simulink model "walking_beam"  (R2026a)
settings: Solver=daessc  StopTime=5  MaxStep=5e-4  RelTol=1e-4
StopFcn:
  | plot_F3_vs_theta2
values from neighbouring files (symbols this model uses):
  s = sign(v)    [plot_F3_vs_theta2.m]
undefined symbols (not defined in the file or in its folder): X, Y, Z
libraries: sm_lib x33, nesl_utility x10, simulink x1
(part 1 of 2)
settings Model: Creator=Admin  LastModifiedBy=Admin
settings SimscapeCC: SimscapeLogType=none
settings ExplorerConfigSet: InternalSimMechanicsExplorerSettings=|
  | <ExplorerConfiguration>
  | 
  |   <canonicalview>default</canonicalview>
  | 
  |   <TilePanel>
  |     <TileInfo>
  |       <Tiles Columns="1" Count="1" Height="706" Rows="1" Width="1316">
  |         <Row Weight="1"/>
  |         <Column Weight="1"/>
  |         <Tile Height="1" Width="1" X="0" Y="0"/>
  |       </Tiles>
  |     </TileInfo>
  |     <SceneInfo>
  |       <SceneViewer>
  |         <IsThisViewStd>
  |           <IsStandardView>off</IsStandardView>
  |           <StandardViewName>Front</StandardViewName>
  |         </IsThisViewStd>
  |         <BGColor>
  |           <R>1</R>
  |           <G>1</G>
  |           <B>1</B>
  |           <A>1</A>
  |         </BGColor>
  |         <Camera>
  |           <DoPerspective>off</DoPerspective>
  |           <Position>
  |             <X>0.069016977308352018</X>
  |             <Y>-0.1702544305806459</Y>
  |             <Z>1.192738584381912</Z>
  |           </Position>
  |           <Center>
  |             <X>0.29948564897094587</X>
  |             <Y>0.074994979776969922</Y>
  |             <Z>0.089914238686012116</Z>
  |           </Center>
  |           <Up>
  |             <X>0.10827439580495295</X>
  |             <Y>0.9653807046978804</Y>
  |             <Z>0.23731150458858177</Z>
  |           </Up>
  |           <XLim>0.16957681948984568</XLim>
  |           <YLim>0.16957681948984568</YLim>
  |           <ViewLimDist>0.01</ViewLimDist>
  |         </Camera>
  |       </SceneViewer>
  |     </SceneInfo>
  |   </TilePanel>
  | 
  |   <MechEditorPanel>
  |     <GfxPanelCameraMap/>
  |     <Cameras/>
  |     <VideoCreator>
  |       <IncludeTiles>All</IncludeTiles>
  |       <IncludeTime>on</IncludeTime>
  |       <IncludeWorldFrame>off</IncludeWorldFrame>
  |       <PlaybackSpeedRatio>1</PlaybackSpeedRatio>
  |       <FrameRate>60</FrameRate>
  |       <FrameSize>auto</FrameSize>
  |       <VideoFormat>MotionJPEGAVI</VideoFormat>
  |     </VideoCreator>
  |   </MechEditorPanel>
  | 
  |   <PlaybackSettings>
  |     <PlaybackSpeedFactor>1</PlaybackSpeedFactor>
  |   </PlaybackSettings>
  | 
  | </ExplorerConfiguration>

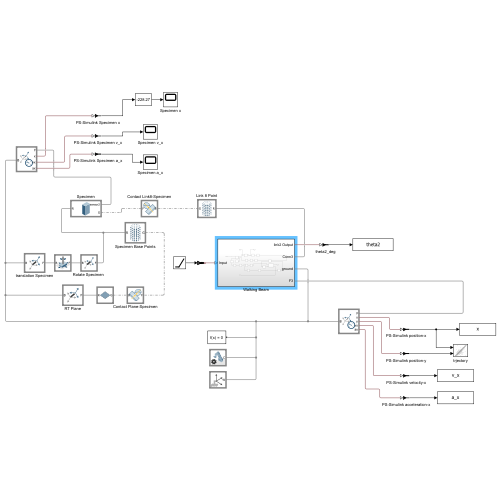
[thumbnail: Simulink's stored preview of the top-level diagram]
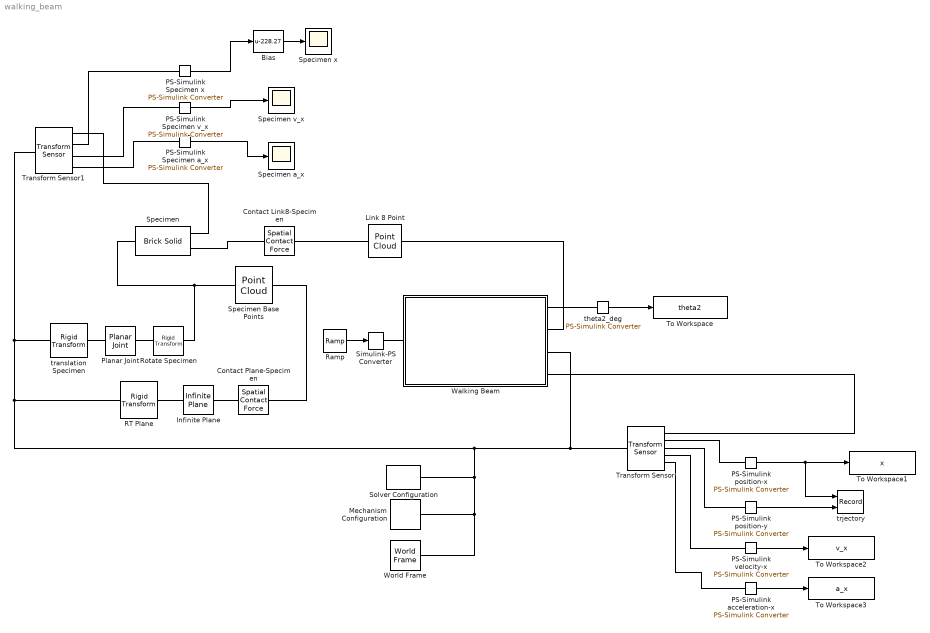
== system walking_beam ==
  Bias : Bias  Bias=-228.27  SaturateOnIntegerOverflow=off
  Contact Link8-Specimen : sm_lib/Forces and Torques/Spatial Contact Force  SenseSeparationDistance=off  NormalForceType=SmoothSpringDamper  NormalStiffness=500  NormalStiffnessUnits=N/m  NormalDamping=1.4  NormalDampingUnits=N/(m/s)  NormalTransitionRegionWidth=1e-05  NormalTransitionRegionWidthUnits=m  FrictionType=SmoothStickSlip  CoefficientOfStaticFriction=0.4  CoefficientOfDynamicFriction=0.3  FrictionalCriticalVelocity=0.001  FrictionalCriticalVelocityUnits=m/s  SenseContactSignal=off  SensePenetrationDepth=off  SenseNormalVelocity=off  SenseTangentialVelocity=off  SensingForceTorqueDirection=BaseOnFollower  SensingForceTorqueResolutionFrame=BaseFrame  SenseNormalForce=off  SenseNormalForceMagnitude=off  SenseNormalTorque=off  SenseFrictionalForce=off  SenseFrictionalForceMagnitude=off  SenseFrictionalTorque=off  SenseTotalForce=off  SenseTotalTorque=off  SenseContactBaseRotation=off  SenseContactBaseTranslation=off  SenseContactFollowerRotation=off  SenseContactFollowerTranslation=off  ZeroCrossDetectContactStartAndEnd=off
  Contact Plane-Specimen : sm_lib/Forces and Torques/Spatial Contact Force  SenseSeparationDistance=off  NormalForceType=SmoothSpringDamper  NormalStiffness=500  NormalStiffnessUnits=N/m  NormalDamping=0.7  NormalDampingUnits=N/(m/s)  NormalTransitionRegionWidth=1e-05  NormalTransitionRegionWidthUnits=m  FrictionType=SmoothStickSlip  CoefficientOfStaticFriction=0.4  CoefficientOfDynamicFriction=0.3  FrictionalCriticalVelocity=0.001  FrictionalCriticalVelocityUnits=m/s  SenseContactSignal=off  SensePenetrationDepth=off  SenseNormalVelocity=off  SenseTangentialVelocity=off  SensingForceTorqueDirection=BaseOnFollower  SensingForceTorqueResolutionFrame=BaseFrame  SenseNormalForce=off  SenseNormalForceMagnitude=off  SenseNormalTorque=off  SenseFrictionalForce=off  SenseFrictionalForceMagnitude=off  SenseFrictionalTorque=off  SenseTotalForce=off  SenseTotalTorque=off  SenseContactBaseRotation=off  SenseContactBaseTranslation=off  SenseContactFollowerRotation=off  SenseContactFollowerTranslation=off  ZeroCrossDetectContactStartAndEnd=off
  Infinite Plane : sm_lib/Curves and Surfaces/Infinite Plane  GraphicType=Rectangle  GraphicPlaneWidth=300  GraphicPlaneWidthUnits=mm  GraphicPlaneHeight=60  GraphicPlaneHeightUnits=mm  GraphicVisPropType=SimpleVisualProperties  GraphicDiffuseColor=[1 1 1]  GraphicOpacity=0  GraphicSpecularColor=[0.5 0.5 0.5 1.0]  GraphicAmbientColor=[0.15 0.15 0.15 1.0]  GraphicEmissiveColor=[0.0 0.0 0.0 1.0]  GraphicShininess=75
  Link 8 Point : sm_lib/Curves and Surfaces/Point Cloud  CoordinatesMatrix=[-16.663 2.5 -98.537;-16.663 2.5 -97.5701;-16.663 2.5 -96.6031;-16.663 2.5 -95.6362;-16.663 2.5 -94.6693;-16.663 2.5 -93.7024;-16.663 2.5 -92.7354;-16.663 2.5 -91.7685;-16.663 2.5 -90.8016;-16.663 2.5 -89.8346;-16.663 2.5 -88.8677;-16.663 2.5 -87.9008;-16.663 2.5 -86.9339;-16.663 2.5 -85.9669;-16.663 2.5 -85;-15.663 2.5 -98.537;-14.663 2.5 -98.537;-14.663 2.5 -97.5701;-14.663 2.5 -96.6031;-14.663 2.5 -95.6362;-14.663 2.5 -94.6693;-14.663 2.5 -93.7024;-14.663 2.5 -92.7354;-14.663 2.5 -91.7685;-14.663 2.5 -90.8016;-14.663 2.5 -89.8346;-14.663 2.5 -88.8677;-14.663 2.5 -87.9008;-14.663 2.5 -86.9339;-14.663 2.5 -85.9669;-14.663 2.5 -85;0.337 2.5 -98.537;0.337 2.5 -97.5701;0.337 2.5 -96.6031;0.337 2.5 -95.6362;0.337 2.5 -94.6693;0.337 2.5 -93.7024;0.337 2.5 -92.7354;0.337 2.5 -91.7685;0.337 2.5 -90.8016;0.337 2.5 -89.8346;0.337 2.5 -88.8677;0.337 2.5 -87.9008;0.337 2.5 -86.9339;0.337 2.5 -85.9669;0.337 2.5 -85;1.337 2.5 -98.537;2.337 2.5 -98.537;2.337 2.5 -97.5701;2.337 2.5 -96.6031;2.337 2.5 -95.6362;2.337 2.5 -94.6693;2.337 2.5 -93.7024;2.337 2.5 -92.7354;2.337 2.5 -91.7685;2.337 2.5 -90.8016;2.337 2.5 -89.8346;2.337 2.5 -88.8677;2.337 2.5 -87.9008;2.337 2.5 -86.9339;2.337 2.5 -85.9669;2.337 2.5 -85;17.337 2.5 -98.537;17.337 2.5 -97.5701;17.337 2.5 -96.6031;17.337 2.5 -95.6362;17.337 2.5 -94.6693;17.337 2.5 -93.7024;17.337 2.5 -92.7354;17.337 2.5 -91.7685;17.337 2.5 -90.8016;17.337 2.5 -89.8346;17.337 2.5 -88.8677;17.337 2.5 -87.9008;17.337 2.5 -86.9339;17.337 2.5 -85.9669;17.337 2.5 -85;18.337 2.5 -98.537;19.337 2.5 -98.537;19.337 2.5 -97.5701;19.337 2.5 -96.6031;19.337 2.5 -95.6362;19.337 2.5 -94.6693;19.337 2.5 -93.7024;19.337 2.5 -92.7354;19.337 2.5 -91.7685;19.337 2.5 -90.8016;19.337 2.5 -89.8346;19.337 2.5 -88.8677;19.337 2.5 -87.9008;19.337 2.5 -86.9339;19.337 2.5 -85.9669;19.337 2.5 -85;34.337 2.5 -98.537;34.337 2.5 -97.5701;34.337 2.5 -96.6031;34.337 2.5 -95.6362;34.337 2.5 -94.6693;34.337 2.5 -93.7024;34.337 2.5 -92.7354;34.337 2.5 -91.7685;34.337 2.5 -90.8016;34.337 2.5 -89.8346;34.337 2.5 -88.8677;34.337 2.5 -87.9008;34.337 2.5 -86.9339;34.337 2.5 -85.9669;34.337 2.5 -85;35.337 2.5 -98.537;36.337 2.5 -98.537;36.337 2.5 -97.5701;36.337 2.5 -96.6031;36.337 2.5 -95.6362;36.337 2.5 -94.6693;36.337 2.5 -93.7024;36.337 2.5 -92.7354;36.337 2.5 -91.7685;36.337 2.5 -90.8016;36.337 2.5 -89.8346;36.337 2.5 -88.8677;36.337 2.5 -87.9008;36.337 2.5 -86.9339;36.337 2.5 -85.9669;36.337 2.5 -85;51.337 2.5 -98.537;51.337 2.5 -97.5701;51.337 2.5 -96.6031;51.337 2.5 -95.6362;51.337 2.5 -94.6693;51.337 2.5 -93.7024;51.337 2.5 -92.7354;51.337 2.5 -91.7685;51.337 2.5 -90.8016;51.337 2.5 -89.8346;51.337 2.5 -88.8677;51.337 2.5 -87.9008;51.337 2.5 -86.9339;51.337 2.5 -85.9669;51.337 2.5 -85;52.337 2.5 -98.537;53.337 2.5 -98.537;53.337 2.5 -97.5701;53.337 2.5 -96.6031;53.337 2.5 -95.6362;53.337 2.5 -94.6693;53.337 2.5 -93.7024;53.337 2.5 -92.7354;53.337 2.5 -91.7685;53.337 2.5 -90.8016;53.337 2.5 -89.8346;53.337 2.5 -88.8677;53.337 2.5 -87.9008;53.337 2.5 -86.9339;53.337 2.5 -85.9669;53.337 2.5 -85;68.337 2.5 -98.537;68.337 2.5 -97.5701;68.337 2.5 -96.6031;68.337 2.5 -95.6362;68.337 2.5 -94.6693;68.337 2.5 -93.7024;68.337 2.5 -92.7354;68.337 2.5 -91.7685;68.337 2.5 -90.8016;68.337 2.5 -89.8346;68.337 2.5 -88.8677;68.337 2.5 -87.9008;68.337 2.5 -86.9339;68.337 2.5 -85.9669;68.337 2.5 -85;69.337 2.5 -98.537;70.337 2.5 -98.537;70.337 2.5 -97.5701;70.337 2.5 -96.6031;70.337 2.5 -95.6362;70.337 2.5 -94.6693;70.337 2.5 -93.7024;70.337 2.5 -92.7354;70.337 2.5 -91.7685;70.337 2.5 -90.8016;70.337 2.5 -89.8346;70.337 2.5 -88.8677;70.337 2.5 -87.9008;70.337 2.5 -86.9339;70.337 2.5 -85.9669;70.337 2.5 -85;85.337 2.5 -98.537;85.337 2.5 -97.5701;85.337 2.5 -96.6031;85.337 2.5 -95.6362;85.337 2.5 -94.6693;85.337 2.5 -93.7024;85.337 2.5 -92.7354;85.337 2.5 -91.7685;85.337 2.5 -90.8016;85.337 2.5 -89.8346;85.337 2.5 -88.8677;85.337 2.5 -87.9008;85.337 2.5 -86.9339;85.337 2.5 -85.9669;85.337 2.5 -85;86.337 2.5 -98.537;87.337 2.5 -98.537;87.337 2.5 -97.5701 ...(+3445 chars)]  CoordinatesMatrixUnits=mm  GraphicType=MarkerCloud  GraphicSphereRadius=0.4  GraphicSphereRadiusUnits=mm  GraphicVisPropType=SimpleVisualProperties  GraphicDiffuseColor=[0.9 0.1 0.1]  GraphicOpacity=1  GraphicSpecularColor=[0.5 0.5 0.5 1.0]  GraphicAmbientColor=[0.15 0.15 0.15 1.0]  GraphicEmissiveColor=[0.0 0.0 0.0 1.0]  GraphicShininess=75
  Mechanism Configuration : sm_lib/Utilities/Mechanism Configuration  UniformGravity=Constant  GravityVector=[0 -9.80665 0]  GravityVectorUnits=m/s^2  LinearizationDelta=0.001  JointModeTransitionNonlinearIterations=2
  PS-Simulink Specimen a_x : nesl_utility/PS-Simulink Converter  PhysicalDomain=network_engine_domain  SubClassName=ps_output  LeftPortType=input  RightPortType=output  PseudoPeriodic=off  Frequencies=[]  VectorFormat=1-D array  Unit=mm/s^2  AffineConversion=off
  PS-Simulink Specimen v_x : nesl_utility/PS-Simulink Converter  PhysicalDomain=network_engine_domain  SubClassName=ps_output  LeftPortType=input  RightPortType=output  PseudoPeriodic=off  Frequencies=[]  VectorFormat=1-D array  Unit=mm/s  AffineConversion=off
  PS-Simulink Specimen x : nesl_utility/PS-Simulink Converter  PhysicalDomain=network_engine_domain  SubClassName=ps_output  LeftPortType=input  RightPortType=output  PseudoPeriodic=off  Frequencies=[]  VectorFormat=1-D array  Unit=mm  AffineConversion=off
  PS-Simulink acceleration-x : nesl_utility/PS-Simulink Converter  PhysicalDomain=network_engine_domain  SubClassName=ps_output  LeftPortType=input  RightPortType=output  PseudoPeriodic=off  Frequencies=[]  VectorFormat=inherit  Unit=mm/s^2  AffineConversion=off
  PS-Simulink position-x : nesl_utility/PS-Simulink Converter  PhysicalDomain=network_engine_domain  SubClassName=ps_output  LeftPortType=input  RightPortType=output  PseudoPeriodic=off  Frequencies=[]  VectorFormat=1-D array  Unit=mm  AffineConversion=off
  PS-Simulink position-y : nesl_utility/PS-Simulink Converter  PhysicalDomain=network_engine_domain  SubClassName=ps_output  LeftPortType=input  RightPortType=output  PseudoPeriodic=off  Frequencies=[]  VectorFormat=1-D array  Unit=mm  AffineConversion=off
  PS-Simulink velocity-x : nesl_utility/PS-Simulink Converter  PhysicalDomain=network_engine_domain  SubClassName=ps_output  LeftPortType=input  RightPortType=output  PseudoPeriodic=off  Frequencies=[]  VectorFormat=inherit  Unit=mm/s  AffineConversion=off
  Planar Joint : sm_lib/Joints/Planar Joint  JointMode=Normal  CompositeWrenchDir=FollowerOnBase  CompositeWrenchFrame=BaseFrame  SenseConstraintForce=off  SenseConstraintTorque=off  SenseTotalForce=off  SenseTotalTorque=off  PxPositionTargetSpecify=on  PxPositionTargetPriority=High  PxPositionTargetValue=228.27  PxPositionTargetValueUnits=mm  PxVelocityTargetSpecify=on  PxVelocityTargetPriority=High  PxVelocityTargetValue=0  PxVelocityTargetValueUnits=m/s  PxEquilibriumPosition=0  PxEquilibriumPositionUnits=m  PxSpringStiffness=0  PxSpringStiffnessUnits=N/m  PxDampingCoefficient=0  PxDampingCoefficientUnits=N/(m/s)  PxLowerLimitSpecify=off  PxLowerLimitBound=-1  PxLowerLimitBoundUnits=m  PxLowerLimitStiffness=1e6  PxLowerLimitStiffnessUnits=N/m  PxLowerLimitDamping=1e3  PxLowerLimitDampingUnits=N/(m/s)  PxLowerLimitTransitionRegionWidth=1e-4  PxLowerLimitTransitionRegionWidthUnits=m  PxUpperLimitSpecify=off  PxUpperLimitBound=1  PxUpperLimitBoundUnits=m  PxUpperLimitStiffness=1e6  PxUpperLimitStiffnessUnits=N/m  PxUpperLimitDamping=1e3  PxUpperLimitDampingUnits=N/(m/s)  PxUpperLimitTransitionRegionWidth=1e-4  PxUpperLimitTransitionRegionWidthUnits=m  PxTorqueActuationMode=NoTorque  PxMotionActuationMode=ComputedMotion  PxSensePosition=off  PxSenseVelocity=off  PxSenseAcceleration=off  PxSenseTorqueForce=off  PxSenseLowerLimitTorqueForce=off  PxSenseUpperLimitTorqueForce=off  PyPositionTargetSpecify=on  PyPositionTargetPriority=High  PyPositionTargetValue=187.1  PyPositionTargetValueUnits=mm  PyVelocityTargetSpecify=on  PyVelocityTargetPriority=High  PyVelocityTargetValue=0  PyVelocityTargetValueUnits=m/s  PyEquilibriumPosition=0  PyEquilibriumPositionUnits=m  PySpringStiffness=0  PySpringStiffnessUnits=N/m  PyDampingCoefficient=0  PyDampingCoefficientUnits=N/(m/s)  PyLowerLimitSpecify=off  PyLowerLimitBound=-1  PyLowerLimitBoundUnits=m  PyLowerLimitStiffness=1e6  PyLowerLimitStiffnessUnits=N/m  PyLowerLimitDamping=1e3  PyLowerLimitDampingUnits=N/(m/s)  PyLowerLimitTransitionRegionWidth=1e-4  PyLowerLimitTransitionRegionWidthUnits=m  PyUpperLimitSpecify=off  PyUpperLimitBound=1  PyUpperLimitBoundUnits=m  PyUpperLimitStiffness=1e6  PyUpperLimitStiffnessUnits=N/m  PyUpperLimitDamping=1e3  PyUpperLimitDampingUnits=N/(m/s)  PyUpperLimitTransitionRegionWidth=1e-4  PyUpperLimitTransitionRegionWidthUnits=m  PyTorqueActuationMode=NoTorque  PyMotionActuationMode=ComputedMotion  PySensePosition=off  PySenseVelocity=off  PySenseAcceleration=off  PySenseTorqueForce=off  PySenseLowerLimitTorqueForce=off  PySenseUpperLimitTorqueForce=off  RzPositionTargetSpecify=on  RzPositionTargetPriority=High  RzPositionTargetValue=0  RzPositionTargetValueUnits=deg  RzVelocityTargetSpecify=on  RzVelocityTargetPriority=High  RzVelocityTargetValue=0  RzVelocityTargetValueUnits=deg/s  RzEquilibriumPosition=0  RzEquilibriumPositionUnits=deg  RzSpringStiffness=0  RzSpringStiffnessUnits=N*m/deg  RzDampingCoefficient=0  RzDampingCoefficientUnits=N*m/(deg/s)  RzLowerLimitSpecify=off  RzLowerLimitBound=-90  RzLowerLimitBoundUnits=deg  RzLowerLimitStiffness=1e4  RzLowerLimitStiffnessUnits=N*m/deg  RzLowerLimitDamping=10  RzLowerLimitDampingUnits=N*m/(deg/s)  RzLowerLimitTransitionRegionWidth=0.1  RzLowerLimitTransitionRegionWidthUnits=deg  RzUpperLimitSpecify=off  RzUpperLimitBound=90  RzUpperLimitBoundUnits=deg  RzUpperLimitStiffness=1e4  RzUpperLimitStiffnessUnits=N*m/deg  RzUpperLimitDamping=10  RzUpperLimitDampingUnits=N*m/(deg/s)  RzUpperLimitTransitionRegionWidth=0.1  RzUpperLimitTransitionRegionWidthUnits=deg  RzTorqueActuationMode=NoTorque  RzMotionActuationMode=ComputedMotion  RzSensePosition=off  RzSenseVelocity=off  RzSenseAcceleration=off  RzSenseTorqueForce=off  RzSenseLowerLimitTorqueForce=off  RzSenseUpperLimitTorqueForce=off
  RT Plane : sm_lib/Frames and Transforms/Rigid Transform  RotationMethod=StandardAxis  FollAlignAxisA=+X  BaseAlignAxisA=+Y  FollAlignAxisB=+Y  BaseAlignAxisB=+Z  RotationStandardAxis=+X  RotationAngle=-90  RotationAngleUnits=deg  RotationArbitraryAxis=[0 0 1]  RotationSequenceAxes=FollowerAxes  RotationSequence=XYX  RotationSequenceAngles=[0 0 0]  RotationSequenceAnglesUnits=deg  RotationMatrix=[1 0 0;0 1 0;0 0 1]  Quaternion=[1 0 0 0]  TranslationMethod=Cartesian  TranslationCartesianOffset=[228.27 184.6 128.77]  TranslationCartesianOffsetUnits=mm  TranslationStandardAxis=+Z  TranslationStandardOffset=0  TranslationStandardOffsetUnits=m  TranslationROffset=0  TranslationROffsetUnits=m  TranslationThetaOffset=0  TranslationThetaOffsetUnits=deg  TranslationZOffset=0  TranslationZOffsetUnits=m
  Ramp : simulink/Sources/Ramp  slope=10  start=0  InitialOutput=10
  "Rotate Specimen " : sm_lib/Frames and Transforms/Rigid Transform  RotationMethod=StandardAxis  FollAlignAxisA=+X  BaseAlignAxisA=+Y  FollAlignAxisB=+Y  BaseAlignAxisB=+Z  RotationStandardAxis=+X  RotationAngle=90  RotationAngleUnits=deg  RotationArbitraryAxis=[0 0 1]  RotationSequenceAxes=FollowerAxes  RotationSequence=XYX  RotationSequenceAngles=[0 0 0]  RotationSequenceAnglesUnits=deg  RotationMatrix=[1 0 0;0 1 0;0 0 1]  Quaternion=[1 0 0 0]  TranslationMethod=None  TranslationCartesianOffset=[0 0 0]  TranslationCartesianOffsetUnits=m  TranslationStandardAxis=+Z  TranslationStandardOffset=0  TranslationStandardOffsetUnits=m  TranslationROffset=0  TranslationROffsetUnits=m  TranslationThetaOffset=0  TranslationThetaOffsetUnits=deg  TranslationZOffset=0  TranslationZOffsetUnits=m
  Simulink-PS Converter : nesl_utility/Simulink-PS Converter  PhysicalDomain=network_engine_domain  SubClassName=ps_input  LeftPortType=input  RightPortType=output  PseudoPeriodic=off  Frequencies=[]  NoiseDistribution=none  NoiseParameters=[]  Unit=rad  AffineConversion=off  FilteringAndDerivatives=filter  SimscapeFilterOrder=2  InputFilterTimeConstant=0.001  UdotUserProvided=0
  Solver Configuration : nesl_utility/Solver Configuration  PhysicalDomain=network_engine_domain  SubClassName=solver  LeftPortType=input  RightPortType=generic  Tones=[]  Harmonics=[]  SimulateNoise=off  Profile=off  UseLocalSampling=off  EnableSwitchedLinearOptims=on  FrequencyDomain=off  UseCCode=off  RelTol=0.001  AbsTol=0.001  MinStep=1e-09  ToWorkspace=off  RevertToSquareIcSolve=off  NumHomotopyIterations=100  PhasorMode=off  PhasorModeNumHarmonics=1  ConsistencySolver=NEWTON_XTOL_AFTER_FTOL  CanonicalOrdering=CANONICAL  OptimizeIntermediates=OPTIMIZED  IndexReductionMethod=DerivativeReplacement  DoDC=off  ResidualTolerance=1e-09  ConsistencyTolSource=GLOBAL  ConsistencyAbsTol=0.001  ConsistencyRelTol=0.001  ConsistencyTolFactor=0.001  UseLocalSolver=off  LocalSolverChoice=NE_BACKWARD_EULER_ADVANCER  ResolveIndetEquations=on  FunctionEvalNumThread=1  LocalSolverSampleTime=0.001  DoFixedCost=off  MaxNonlinIter=3  MaxModeIter=2  ComputeImpulses=off  ImpulseIterations=2  LinearAlgebra=auto  LinearAlgebraNumThread=0  EquationFormulation=NE_TIME_EF  DelaysMemoryBudget=1024  AutomaticFiltering=on  FilteringTimeConstant=0.001  PartitionStorageMethod=AS_NEEDED  PartitionMemoryBudget=1024  PartitionMethod=ROBUST  MultibodyUseLocalSolver=off  MultibodyLocalSolverChoice=ODE1  MultibodyLocalSolverSampleTime=0.001
  Specimen : sm_lib/Body Elements/Brick Solid  BrickDimensions=[5 30 5]  BrickDimensionsUnits=mm  ExportEntireGeometry=on  InertiaType=CalculateFromGeometry  BasedOnType=Density  Density=1000  DensityUnits=kg/m^3  Mass=1  MassUnits=kg  CenterOfMass=[0 0 0]  CenterOfMassUnits=m  MomentsOfInertia=[1 1 1]  MomentsOfInertiaUnits=kg*m^2  ProductsOfInertia=[0 0 0]  ProductsOfInertiaUnits=kg*m^2  GraphicType=FromGeometry  MarkerShape=Sphere  MarkerSize=10  GraphicVisPropType=SimpleVisualProperties  GraphicDiffuseColor=[0.75 0.65 0.95]  GraphicOpacity=1  GraphicSpecularColor=[0.5 0.5 0.5 1.0]  GraphicAmbientColor=[0.15 0.15 0.15 1.0]  GraphicEmissiveColor=[0.0 0.0 0.0 1.0]  GraphicShininess=75  DoExposeReferenceFrame=on  SerializedFrames=|
      | <Frames>
      | 
      |   <Frame>
      |     <Id>Frame1</Id>
      |     <Value>
      |       <Name>sensor2</Name>
      |       <Origin>
      |         <Source>ReferenceFrame</Source>
      |         <FeatureName></FeatureName>
      |       </Origin>
      |       <PrimaryAxis>
      |         <DefinedDirection>+Z</DefinedDirection>
      |         <Source>ReferenceFrame</Source>
      |         <SourceDirection>+Z</SourceDirection>
      |         <FeatureName></FeatureName>
      |       </PrimaryAxis>
      |       <SecondaryAxis>
      |         <DefinedDirection>+X</DefinedDirection>
      |         <Source>ReferenceFrame</Source>
      |         <SourceDirection>+X</SourceDirection>
      |         <FeatureName></FeatureName>
      |       </SecondaryAxis>
      |     </Value>
      |   </Frame>
      | 
      | </Frames>
  Specimen Base Points : sm_lib/Curves and Surfaces/Point Cloud  CoordinatesMatrix=[-2.5 -10 2.5;2.5 -10 2.5;2.5 10 2.5;-2.5 10 2.5]  CoordinatesMatrixUnits=mm  GraphicType=MarkerCloud  GraphicSphereRadius=0.4  GraphicSphereRadiusUnits=mm  GraphicVisPropType=SimpleVisualProperties  GraphicDiffuseColor=[0.2 0.2 0.9]  GraphicOpacity=1  GraphicSpecularColor=[0.5 0.5 0.5 1.0]  GraphicAmbientColor=[0.15 0.15 0.15 1.0]  GraphicEmissiveColor=[0.0 0.0 0.0 1.0]  GraphicShininess=75
  Specimen a_x : Scope
      settings: ActiveDisplayYMinimum=-128615.45700333494  ActiveDisplayYMaximum=1.0858097042017304E+6  DataLoggingVariableName=ScopeData2
  Specimen v_x : Scope
      settings: ActiveDisplayYMinimum=-17.214449819310651  ActiveDisplayYMaximum=151.84850866140505
  Specimen x : Scope
      settings: ActiveDisplayYMinimum=-28.751888500285233  ActiveDisplayYMaximum=165.83973606812339
  To Workspace : ToWorkspace  VariableName=theta2  SaveFormat=Timeseries  SampleTime=-1
  To Workspace1 : ToWorkspace  VariableName=x  SaveFormat=Timeseries  SampleTime=-1
  To Workspace2 : ToWorkspace  VariableName=v_x  SaveFormat=Timeseries  SampleTime=-1
  To Workspace3 : ToWorkspace  VariableName=a_x  SaveFormat=Timeseries  SampleTime=-1
  Transform Sensor : sm_lib/Frames and Transforms/Transform Sensor  MeasurementFrame=World  RotationSequence=XYX  SenseAngle=off  SenseAxis=off  SenseQ=off  SenseR=off  SenseRotationSequence=off  SenseOmegaX=off  SenseOmegaY=off  SenseOmegaZ=off  SenseOmega=off  SenseQDot=off  SenseRDot=off  SenseRotationSequenceDot=off  SenseAlphaX=off  SenseAlphaY=off  SenseAlphaZ=off  SenseAlpha=off  SenseQDDot=off  SenseRDDot=off  SenseX=on  SenseY=on  SenseZ=off  SenseXYZ=off  SenseRad=off  SenseAzim=off  SenseDist=off  SenseInc=off  SenseXDot=on  SenseYDot=off  SenseZDot=off  SenseXYZDot=off  SenseRadDot=off  SenseAzimDot=off  SenseDistDot=off  SenseIncDot=off  SenseXDDot=on  SenseYDDot=off  SenseZDDot=off  SenseXYZDDot=off  SenseRadDDot=off  SenseAzimDDot=off  SenseDistDDot=off  SenseIncDDot=off
  Transform Sensor1 : sm_lib/Frames and Transforms/Transform Sensor  MeasurementFrame=World  RotationSequence=XYX  SenseAngle=off  SenseAxis=off  SenseQ=off  SenseR=off  SenseRotationSequence=off  SenseOmegaX=off  SenseOmegaY=off  SenseOmegaZ=off  SenseOmega=off  SenseQDot=off  SenseRDot=off  SenseRotationSequenceDot=off  SenseAlphaX=off  SenseAlphaY=off  SenseAlphaZ=off  SenseAlpha=off  SenseQDDot=off  SenseRDDot=off  SenseX=on  SenseY=off  SenseZ=off  SenseXYZ=off  SenseRad=off  SenseAzim=off  SenseDist=off  SenseInc=off  SenseXDot=on  SenseYDot=off  SenseZDot=off  SenseXYZDot=off  SenseRadDot=off  SenseAzimDot=off  SenseDistDot=off  SenseIncDot=off  SenseXDDot=on  SenseYDDot=off  SenseZDDot=off  SenseXYZDDot=off  SenseRadDDot=off  SenseAzimDDot=off  SenseDistDDot=off  SenseIncDDot=off
  Walking Beam : Subsystem
  World Frame : sm_lib/Frames and Transforms/World Frame
  theta2_deg : nesl_utility/PS-Simulink Converter  PhysicalDomain=network_engine_domain  SubClassName=ps_output  LeftPortType=input  RightPortType=output  PseudoPeriodic=off  Frequencies=[]  VectorFormat=1-D array  Unit=deg  AffineConversion=off
  translation Specimen : sm_lib/Frames and Transforms/Rigid Transform  RotationMethod=None  FollAlignAxisA=+X  BaseAlignAxisA=+Y  FollAlignAxisB=+Y  BaseAlignAxisB=+Z  RotationStandardAxis=+Z  RotationAngle=0  RotationAngleUnits=deg  RotationArbitraryAxis=[0 0 1]  RotationSequenceAxes=FollowerAxes  RotationSequence=XYX  RotationSequenceAngles=[0 0 0]  RotationSequenceAnglesUnits=deg  RotationMatrix=[1 0 0;0 1 0;0 0 1]  Quaternion=[1 0 0 0]  TranslationMethod=Cartesian  TranslationCartesianOffset=[0 0 128.77]  TranslationCartesianOffsetUnits=mm  TranslationStandardAxis=+Z  TranslationStandardOffset=0  TranslationStandardOffsetUnits=m  TranslationROffset=0  TranslationROffsetUnits=m  TranslationThetaOffset=0  TranslationThetaOffsetUnits=deg  TranslationZOffset=0  TranslationZOffsetUnits=m
  trjectory : Record  NumPorts=2.0  FileSettingsInternal="{\"entries\":[{\"content\":{\"excelSettings\":{\"content\":{},\"type\":\"Streamout.ExcelSettings\"},\"parquetSettings\":{\"content\":{},\"type\":\"Streamout.ParquetSettings\"}},\"type\":\"Streamout.FileSettingStorage\",\"uuid\":\"\"}],\"packageUris\":[\"http:\\/\\/schema.mathworks.com\\/mf0\\/streamout_blocks\\/R2020a\"],\"version\":\"1.0\"}"  FrameSettings=[0, 0]  Layout=[1 1]  SignalsInternal="{\"entries\":[{\"content\":{\"signals\":[{\"content\":{\"blockPath\":[],\"dimensions\":[1],\"domain\":\"\",\"lineColor\":\"#fe330a\",\"lineWidth\":2,\"plots\":[ 1 ],\"port\":1,\"sid\":[\"\"],\"signalID\":1,\"signalName\":\"PS-Simulink position-x\"},\"type\":\"RecordBlkView.Signal\",\"uuid\":\"\"},{\"content\":{\"blockPath\":[],\"dimensions\":[1],\"domain\":\"\",\"lineColor\":\"#139fff\",\"plots\":[ 1 ],\"port\":2,\"sid\":[\"\"],\"signalID\":2,\"signalName\":\"PS-Simulink position-y\"},\"type\":\"RecordBlkView.Signal\",\"uuid\":\"\"}]},\"type\":\"RecordBlkView.InputSignals\",\"uuid\":\"\"}],\"packageUris\":[\"http:\\/\\/schema.mathworks.com\\/mf0\\/streamout_blocks\\/R2020a\"],\"version\":\"1.0\"}"  VisualizationBindings="{\"xyplotplugin\":{\"info\":[{\"series\":[{\"bindingParametersList\":[{\"parameter\":\"X-Axis\",\"signalID\":1,\"signalName\":\"PS-Simulink position-x\"},{\"parameter\":\"Y-Axis\",\"signalID\":2,\"signalName\":\"PS-Simulink position-y\"}],\"seriesID\":0}],\"subplotID\":1}]}}"  CompatibilityTag=XY
  wires:
  Ramp/1 -> Simulink-PS Converter/1
  PS-Simulink position-x/1 -> To Workspace1/1, trjectory/1
  PS-Simulink position-y/1 -> trjectory/2
  theta2_deg/1 -> To Workspace/1
  PS-Simulink velocity-x/1 -> To Workspace2/1
  PS-Simulink acceleration-x/1 -> To Workspace3/1
  PS-Simulink Specimen x/1 -> Bias/1
  PS-Simulink Specimen v_x/1 -> Specimen v_x/1
  PS-Simulink Specimen a_x/1 -> Specimen a_x/1
  Bias/1 -> Specimen x/1
  connections:
  Solver Configuration/RConn1 -- Walking Beam/RConn3 -- Transform Sensor/LConn1 -- Transform Sensor1/LConn1 -- translation Specimen/LConn1 -- RT Plane/LConn1 -- World Frame/RConn1 -- Mechanism Configuration/RConn1
  PS-Simulink position-x/LConn1 -- Transform Sensor/RConn2
  Transform Sensor/RConn3 -- PS-Simulink position-y/LConn1
  Transform Sensor/RConn4 -- PS-Simulink velocity-x/LConn1
  Transform Sensor/RConn5 -- PS-Simulink acceleration-x/LConn1
  RT Plane/RConn1 -- Infinite Plane/LConn1
  translation Specimen/RConn1 -- Planar Joint/LConn1
  Link 8 Point/RConn1 -- Contact Link8-Specimen/LConn1
  Specimen/LConn2 -- Contact Link8-Specimen/RConn1
  Infinite Plane/RConn1 -- Contact Plane-Specimen/LConn1
  Specimen Base Points/RConn1 -- Contact Plane-Specimen/RConn1
  Planar Joint/RConn1 -- "Rotate Specimen "/LConn1
  "Rotate Specimen "/RConn1 -- Specimen/RConn1 -- Specimen Base Points/LConn1
  Walking Beam/LConn1 -- Simulink-PS Converter/RConn1
  Walking Beam/RConn1 -- theta2_deg/LConn1
  Walking Beam/RConn2 -- Link 8 Point/LConn1
  Walking Beam/RConn4 -- Transform Sensor/RConn1
  Specimen/LConn1 -- Transform Sensor1/RConn1
  Transform Sensor1/RConn2 -- PS-Simulink Specimen x/LConn1
  Transform Sensor1/RConn3 -- PS-Simulink Specimen v_x/LConn1
  Transform Sensor1/RConn4 -- PS-Simulink Specimen a_x/LConn1
